simulink model "MPPT_Son"  (R2025a)
settings: Solver=VariableStepAuto  StartTime=0.0  StopTime=7  RelTol=1e-3
libraries: spsSeriesRLCBranchLib x4, simulink x3, spsVoltageMeasurementLib x2, spsCurrentMeasurementLib x1, spsDiodeLib x1, spsMosfetLib x1, spsPVArrayLib x1, spspowerguiLib x1
settings Model: Creator=BORA  LastModifiedBy=BORA

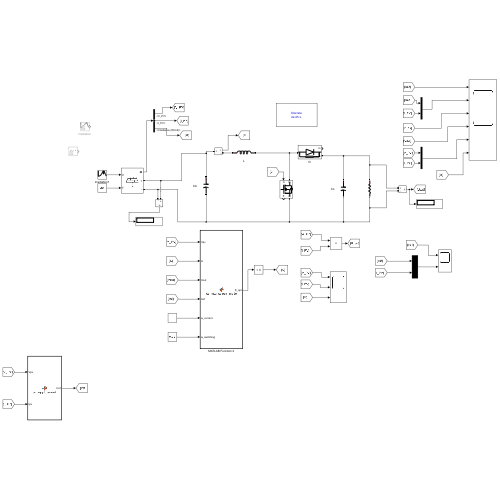
[thumbnail: Simulink's stored preview of the top-level diagram]
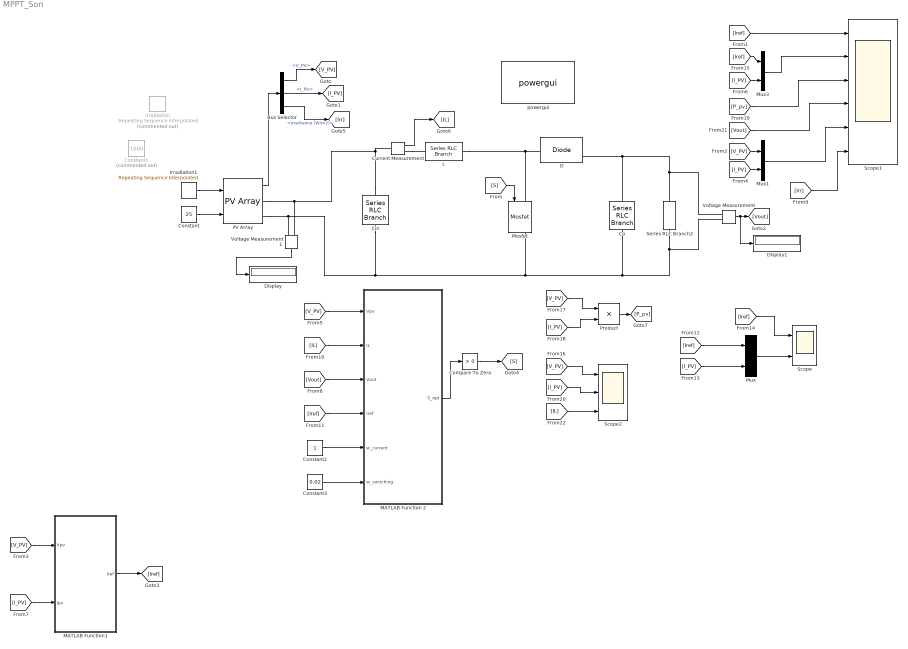
== system MPPT_Son ==
  Bus Selector : BusSelector  OutputSignals=V_PV,I_PV,Irradiance (W/m2)
  Cin : spsSeriesRLCBranchLib/Series RLC Branch  LConnTagsString=__new0  RConnTagsString=__new0  BranchType=C  Resistance=1  Inductance=1e-3  SetiL0=off  InitialCurrent=0  Capacitance=1000e-6  Setx0=off  InitialVoltage=0  Measurements=None
  Co : spsSeriesRLCBranchLib/Series RLC Branch  LConnTagsString=__new0  RConnTagsString=__new0  BranchType=C  Resistance=1  Inductance=1e-3  SetiL0=off  InitialCurrent=0  Capacitance=1000e-6  Setx0=off  InitialVoltage=0  Measurements=None
  Compare To Zero : simulink/Logic and Bit Operations/Compare To Zero  relop=>  OutDataTypeStr=boolean
  Constant : Constant  Value=25
  Constant1 : Constant  Commented=on  Value=1000
  Constant2 : Constant
  Constant3 : Constant  Value=0.02
  Current Measurement : spsCurrentMeasurementLib/Current Measurement  PhasorSimulation=off  OutputType=Complex  PSBequivalent=0
  D : spsDiodeLib/Diode  Ron=0.001  Lon=0  Vf=0.8  IC=0  UseSnubber=0  Rs=500  Cs=250e-9  Measurements=on
  Display : Display
  Display1 : Display
  L : spsSeriesRLCBranchLib/Series RLC Branch  LConnTagsString=__new0  RConnTagsString=__new0  BranchType=L  Resistance=1  Inductance=5e-3  SetiL0=off  InitialCurrent=0  Capacitance=1e-6  Setx0=off  InitialVoltage=0  Measurements=None
  MATLAB Function 2 : MATLAB Function  TreatAsAtomicUnit=on
  MATLAB Function1 : MATLAB Function  TreatAsAtomicUnit=on  SystemSampleTime=110e-6
  Mosfet : spsMosfetLib/Mosfet  Ron=0.001  Lon=0  Rd=0.001  Vfd=0  IC=0  Rs=1e5  Cs=inf  Measurements=on
  Mux : Mux  Inputs=2
  Mux1 : Mux  Inputs=2
  Mux3 : Mux  Inputs=2
  PV Array : spsPVArrayLib/PV Array  Npar=2  Nser=2  PlotType=array @ 25 deg.C & specified irradiances  S_vec=[ 1000 800 600 400 200 ]  Temp_C_vec="[ 45 25  ]"  ModuleName=A10Green Technology A10J-S72-175  PlotWhenSelected=off  Pm=175.0914  Ncell=72  Voc=43.99  Isc=5.17  Vm=36.63  Im=4.78  beta_Voc_pc=-0.3616  alpha_Isc_pc=0.041509  beta_Voc=-0.15907  alpha_Isc=0.002146  IL=5.178  I0=1.7842e-10  nI=0.98852  Rsh=249.6758  Rs=0.38412  RobustModel=off  RobustCellTemperature=313.3991  BAL=on  Tc=1e-6  Tfilter=5e-5
  Product : Product
  Scope : Scope  NumInputPorts=2
      settings: ActiveDisplayYMinimum=-1.1637499999999794  ActiveDisplayYMaximum=10.973749999999816
  Scope1 : Scope  NumInputPorts=6
      settings: TimeSpan=1  ActiveDisplayYMinimum=-1.1787499999999791  ActiveDisplayYMaximum=11.108749999999814
  Scope2 : Scope  NumInputPorts=3
      settings: ActiveDisplayYMinimum=-1  ActiveDisplayYMaximum=1  DataLoggingVariableName=ScopeData2
  Series RLC Branch2 : spsSeriesRLCBranchLib/Series RLC Branch  LConnTagsString=__new0  RConnTagsString=__new0  BranchType=R  Resistance=30  Inductance=1e-3  SetiL0=off  InitialCurrent=0  Capacitance=1e-6  Setx0=off  InitialVoltage=0  Measurements=None
  Voltage Measurement : spsVoltageMeasurementLib/Voltage Measurement  PhasorSimulation=off  OutputType=Complex  PSBequivalent=0
  Voltage Measurement1 : spsVoltageMeasurementLib/Voltage Measurement  PhasorSimulation=off  OutputType=Complex  PSBequivalent=0
  irradiation : simulink/Sources/Repeating Sequence Interpolated  Commented=on  OutValues="[77.3  151.9  260.4  349.3  420.4  538.5  613.1  709.1  623.4  314.7  174.3].'"  TimeValues=[0 0.5 0.75 1.25 1.75 2.19 2.73 3.35 3.42 4.01 4.38].'  LookUpMeth=Interpolation-Use End Values  tsamp=0.001  OutMin=[]  OutMax=[]  OutDataTypeStr=double  OutputDataTypeScalingMode=double  OutDataType=fixdt(0,8)  OutScaling=2^-10
  irradiation1 : simulink/Sources/Repeating Sequence Interpolated  OutValues=[150 200 400 600 800 1000 500 500 1000 800 600 400 200 ].'  TimeValues=[0 1 2.5 3 3.5 4 4.03 4.5 4.53 5 5.5 6 6.5].'  LookUpMeth=Interpolation-Use End Values  tsamp=0.01  OutMin=[]  OutMax=[]  OutDataTypeStr=double  OutputDataTypeScalingMode=double  OutDataType=fixdt(0,8)  OutScaling=2^-10
  powergui : spspowerguiLib/powergui  Priority=1  SimulationMode=Discrete  SampleTime=20e-06  frequency=60  Iterations=50  frequencyindice=0  Pbase=100e6  ErrMax=1e-4  UnitsV=kV  UnitsW=MW  buscounter=0  FunctionMessages=off  echomessages=off  EnableUseOfTLC=off  CurrentSourceSwitches=off  DisableSnubberDevices=off  DisableRonSwitches=off  DisableVfSwitches=off  DisplayEquations=off  AutomaticDiscreteSolvers=off  SolverType=Tustin/Backward Euler (TBE)  Interpol=off  ExternalGateDelay=off  methode=off  Ts=100  x0status=blocks  SPID=on  SwTol=0  HookPort=off  NonlinearTolerance=1e-4  nMaxIteration=100  ContinueOnMaxIteration=off  RestoreLinks=warning  ResistiveCurrentMeasurement=off  Frange=[0:2:500]  Ylog=off  Xlog=on  ShowGrid=off  save=off  variable=ZData  structure=0  ZoomFFT=off  StartTime=0.0  cycles=1  DisplayStyle=1  fundamental=60  FreqAxis=off  MaxFrequency=1000  frequencyindicesteady=1  RmsSteady=1  display=off
  wires:
  irradiation1/1 -> PV Array/1
  [V_PV] -> Product/1
  Voltage Measurement1/1 -> Display/1
  MATLAB Function1/1(Iref) -> [Iref]
  [V_PV] -> MATLAB Function1/1(Vpv)
  Constant/1 -> PV Array/2
  Mux1/1 -> Scope1/5
  Constant3/1 -> MATLAB Function 2/6(w_switching)
  Compare To Zero/1 -> [S]
  [Iref] -> MATLAB Function 2/4(Iref)
  [IL] -> MATLAB Function 2/2(IL)
  [I_PV] -> Product/2
  [Vout] -> MATLAB Function 2/3(Vout)
  [I_PV] -> Mux3/2
  Constant2/1 -> MATLAB Function 2/5(w_current)
  PV Array/1 -> Bus Selector/1
  [I_PV] -> Mux1/2
  [S] -> Mosfet/1
  [Iref] -> Mux3/1
  Voltage Measurement/1 -> Display1/1, [Vout]
  [Vout] -> Scope1/4
  Current Measurement/1 -> [IL]
  [Iref] -> Scope1/1
  [P_pv] -> Scope1/3
  Product/1 -> [P_pv]
  [I_PV] -> MATLAB Function1/2(Ipv)
  Bus Selector/2 -> [I_PV]  "<I_PV>"
  [V_PV] -> Mux1/1
  MATLAB Function 2/1(S_opt) -> Compare To Zero/1
  [V_PV] -> MATLAB Function 2/1(Vpv)
  Bus Selector/1 -> [V_PV]  "<V_PV>"
  Mux3/1 -> Scope1/2
  Bus Selector/3 -> [Irr]  "<Irradiance (W/m2)>"
  [Irr] -> Scope1/6
  [I_PV] -> Mux/2
  [Iref] -> Mux/1
  Mux/1 -> Scope/2
  [Iref] -> Scope/1
  [I_PV] -> Scope2/2
  [V_PV] -> Scope2/1
  [IL] -> Scope2/3
  connections:
  Co/LConn1 -- D/RConn1 -- Voltage Measurement/LConn1 -- Series RLC Branch2/LConn1
  PV Array/RConn2 -- Series RLC Branch2/RConn1 -- Voltage Measurement/LConn2 -- Co/RConn1 -- Mosfet/RConn1 -- Cin/RConn1 -- Voltage Measurement1/LConn2
  Mosfet/LConn1 -- D/LConn1 -- L/RConn1
  Cin/LConn1 -- Current Measurement/LConn1 -- PV Array/RConn1 -- Voltage Measurement1/LConn1
  Current Measurement/RConn1 -- L/LConn1

== matlab function MPPT_Son/MATLAB Function1 ==
  data: Vpv input; Iref output; Ipv input
% function Iref = po_mppt_current(Vpv, Ipv)
%     %#codegen
% 
%     % Nominal başlangıç tahmini (Sadece ilk adımda algoritmayı ayağa kaldırmak için)
%     Imp_nominal = 2;    
%     dI_step     = 0.01; % Her adımda akımı 10 mA değiştir (Çok hassas arama)
% 
%     persistent P_old I_old Iref_prev;
% 
%     if isempty(P_old)
%         I_old     = 0;
%         P_old     = 0;
%         Iref_prev = Imp_nominal; 
%     end
% 
%     Ppv = Vpv * Ipv;   % O anki güç (W)
%     dP  = Ppv - P_old; % Güçteki değişim
%     dI  = Ipv - I_old; % Akımdaki değişim
% 
%     % P&O Akım Yönü Mantığı
%     if dP ~= 0
%         if dP > 0
%             if dI > 0
%                 Iref = Iref_prev + dI_step; % Güç artıyor, akım artıyor -> Devam et
%             else
%                 Iref = Iref_prev - dI_step; % Güç artıyor, akım azalıyor -> Devam et
%             end
%         else
%             if dI > 0
%                 Iref = Iref_prev - dI_step; % Güç azalıyor, akım artıyor -> Geri dön
%             else
%                 Iref = Iref_prev + dI_step; % Güç azalıyor, akım azalıyor -> Geri dön
%             end
%         end
%     else
%         Iref = Iref_prev;
%     end    
% 
%     %% 5. DİNAMİK GÜVENLİK SINIRLANDIRMASI (Saturation)
%     % Sabit Isc yerine o an ölçülen panel akımını (Ipv) baz alıyoruz.
%     % Akım referansı, o anki ölçülen akımın %15'inden fazla yukarısını hedefleyemesin.
%     % Böylece panel o anki ışınımda verebileceğinin ötesine zorlanmaz, voltaj çökmez.
%     I_ust_sinir = Ipv * 1.15; 
% 
%     if Iref > I_ust_sinir
%         Iref = I_ust_sinir; 
%     elseif Iref < 0.5
%         Iref = 0.5; % Akımın tamamen sıfıra kilitlenmesini engelle
%     end
% 
%     %% 6. BİR SONRAKI ADIM İÇİN HAFIZAYI GÜNCELLEME
%     P_old     = Ppv;
%     I_old     = Ipv;
%     Iref_prev = Iref;
% end
% 


    function Iref = po_mppt_current(Vpv, Ipv)

    dI_step = 0.01; % Her adımda akımı 10 mA değiştir

    persistent P_old I_old Iref_prev;

    if isempty(P_old)
        I_old     = Ipv; % İlk adımda ölçülen gerçek akımı hafızaya al
        P_old     = Vpv * Ipv; % İlk adımdaki gerçek gücü hafızaya al
        Iref_prev = Ipv; % Arama başlangıç noktasını doğrudan o anki panel akımı yap!
    end

    Ppv = Vpv * Ipv;   % O anki güç (W)
    dP  = Ppv - P_old; % Güçteki değişim
    dI  = Ipv - I_old; % Akımdaki değişim

    % P&O Akım Yönü Mantığı
    if dP ~= 0
        if dP > 0
            if dI > 0
                Iref = Iref_prev + dI_step;
            else
                Iref = Iref_prev - dI_step;
            end
        else
            if dI > 0
                Iref = Iref_prev - dI_step;
            else
                Iref = Iref_prev + dI_step;
            end
        end
    else
        Iref = Iref_prev;
    end    

    %% 5. ESNEK VE GÜVENLİ GERÇEKÇİ SINIRLANDIRMA
    % Sabit bir Isc belirtmiyoruz. Sadece akımın negatif bölgelere (0'ın altına) 
    % düşmesini engellemek için alt sınır koyuyoruz. Üst sınırı ise tamamen serbest bırakıyoruz.
    if Iref < 0.05
        Iref = 0.05; 
    end

    %% 6. BİR SONRAKI ADIM İÇİN HAFIZAYI GÜNCELLEME
    P_old     = Ppv;
    I_old     = Ipv;
    Iref_prev = Iref;
    end






% 
%     function iref = po_mppt_flowchart(Vpv, Ipv)
%     %#codegen
% 
%     %% 1. ALGORİTMA PARAMETRELERİ (Diyagramdaki Değişkenler)
%     % Şemadaki delta (Delta) akım adım boyunu temsil eder.
%     delta       = 0.01;   
% 
%     persistent P_old V_old iref_prev;
% 
%     % Dinamik Başlangıç Ayarı (Kilitlenmeyi önlemek için ilk ölçümü hafızaya alıyoruz)
%     if isempty(P_old)
%         V_old     = Vpv;
%         P_old     = Vpv * Ipv;
%         iref_prev = Ipv;   % Arama başlangıcını doğrudan anlık panel akımı yapıyoruz
%     end
% 
%     %% 2. HESAPLAMA KATMANI (Diyagramdaki "Calculate" Bloğu)
%     P_k = Vpv * Ipv;       % P(k) = Vin(k) * I(k)
%     dp  = P_k - P_old;     % Delta p = P(k) - P(k-1)
%     dv  = Vpv - V_old;     % Delta v = Vin(k) - Vin(k-1)
% 
%     %% 3. KARAR MEKANİZMASI (Diyagramdaki İki Aşamalı Baklava Dilimleri)
% 
%     % İlk Karar: Delta p > 0 kontrolü
%     if dp > 0
%         % Sol Taraf: Delta p > 0 "yes" yolu
%         if dv > 0
%             % Delta v > 0 "yes"
%             iref = iref_prev + delta;
%         else
%             % Delta v > 0 "no" (yani dv <= 0)
%             iref = iref_prev - delta;
%         end
%     else
%         % Sağ Taraf: Delta p > 0 "no" yolu (yani dp <= 0)
%         % Akış şemasındaki sağdaki baklava dilimi: Delta v < 0 kontrolü
%         if dv < 0
%             % Delta v < 0 "yes"
%             iref = iref_prev - delta;
%         else
%             % Delta v < 0 "no" (yani dv >= 0)
%             iref = iref_prev + delta;
%         end
%     end    
% 
%     %% 4. GÜVENLİK SINIRLANDIRMASI (Saturation)
%     % Akımın negatif bölgelere kaymasını engellemek için sadece esnek bir alt sınır
%     if iref < 0.05
%         iref = 0.05; 
%     end
% 
%     %% 5. HAFIZA GÜNCELLEME (Bir Sonraki Adım İçin k-1 Değerleri)
%     P_old     = P_k;
%     V_old     = Vpv;
%     iref_prev = iref;
% end

== matlab function MPPT_Son/MATLAB Function 2 ==
  data: Vpv input; IL input; Vout input; S_opt output; Iref input; w_current input; w_switching input
function S_opt = fcs_mpc_current_mode(Vpv, IL, Vout, Iref, w_current, w_switching)
    
    
    % 1. SİSTEM PARAMETRELERİ
    L  = 5e-3;   % Boost Bobini (500 uH)
    Ts = 20e-6;    % Örnekleme Zamanı (10 mikrosaniye)
    
    % 2. AĞIRLIK KATSAYILARI
    % w_current   = 2.0;   % Akım takibi ana hedefimiz
    % w_switching = 0.07;  % Anahtarlama sıklığı cezası
    
    persistent S_old;
    if isempty(S_old)
        S_old = 0;
    end
    
    min_cost = inf;
    S_opt = 0;
    
    % 3. OPTİMİZASYON DÖNGÜSÜ
    for S_test = 0:1
        
        % S_test durumuna göre (k+1) adımı Bobin Akımı tahmini (İleri Euler)
        IL_next = IL + (Ts / L) * (Vpv - (1 - S_test) * Vout);
        
        % Yeni Maliyet Fonksiyonu (Sadece Akım Takibi ve Anahtarlama Cezası)
        cost = w_current   * (Iref - IL_next)^2 + w_switching * abs(S_test - S_old);
        
        if cost < min_cost
            min_cost = cost;
            S_opt = S_test;
        end
    end
    
    S_old = S_opt;
end
